simulink model "reachout_demo_PERTURB"  (R2013a)
settings: Solver=ode4  SolverMode=SingleTasking  StartTime=0.0  StopTime=inf  FixedStep=0.0005  RelTol=1e-3
StartFcn:
  |  warndlg('Dexterit-E models cannot run under simulation. Please compile your model and run it from within Dexterit-E.');set_param(bdroot,'SimulationCommand','stop')
model workspace (MAT data in the model file):
  col_x = 1
  col_y = 2
  RADIUS_VIS = 3
  RADIUS_LOG = 4
  COLOR_INIT = 5
  COLOR_REACH = 6
  START_TARGET_COL = 1
  END_TARGET_COL = 7
  LOAD_COL = 8
  DELAY_HAND_FDBK_ON_COL = 11
  MAXREACHTIME_COL = 14
  DELAY_POSTTRIAL_COL = 16
  HAND_FDBK_CNTL_COL = 17
  E_HAND_FDBK_ON = 10
  E_HAND_FDBK_OFF = 11
  WAIT_AT_1stTARGET_COL = 12
  RNDM_WAIT_AT_1stTARGET_COL = 13
  WAIT_AT_2ndTARGET_COL = 15
  X_COL = 1
  Y_COL = 2
  RISE_FALL_COL = 3
  DURATION_COL = 4
  BKIN_STEP_TIME = 0.0005
  TARGET_LABEL = 7
  LABEL_COLOR = 8
  LABEL_SIZE = 9
  GRASP_TARGET = 10
  N_TO_M_GRASP_TAR = 1
  WARNING_COL = 4
  START_FLAG_COL = 6
  TITLE_COL = 5
  E_HOLD_FORCE_1 = 1
  E_HOLD_FORCE_2 = 2
  E_HOLD_1_SUCCESS = 3
  E_HOLD_2_SUCCESS = 4
  E_HOLD_1_FAIL = 5
  E_HOLD_2_FAIL = 6
  E_FORCE_1_LARGER = 7
  E_FORCE_2_LARGER = 8
  E_NOT_HOLDING = 9
  ANSWER_FORCE_1_COL = 2
  ANSWER_FORCE_2_COL = 3
  TIME_TO_ANSWER_COL = 18
  TIME_TO_FAILURE_COL = 19
  CURSOR_OPACITY = 2
  LOAD_1_MAG_COL = 9
  LOAD_2_MAG_COL = 10
  E_LOAD_MAG_1_FIRST = 12
  E_LOAD_MAG_2_FIRST = 13
  GRASP_TARGET_TOLERANCE = 11
undefined symbols (not defined in the file or in its folder): slselsubs
libraries: xpclib x6, Video x6, General x3, KINARM_EP_loads x2, KINARM_general x2, KINARM_IO x1, KINARM_loads x1
CloseFcn:
  | rtwprivate ssgencode ModelCloseRequest b2lab2d
settings Model: ModifiedComment=chris -- Wed Feb 16 09:18:30 2005 -- Version 1.1384  ModifiedHistory=Feb 16/05 - Add error repeat, add offset ramp  ExtModeArmWhenConnect=off  ExtModeLogAll=off  BufferReuse=off  Creator=Chris Grebeldinger  LastModifiedBy=BKIN TECHNOLOGIES
settings DataIOCC: LimitDataPoints=off  SignalLoggingSaveFormat=ModelDataLogs  SaveOutput=off  SaveTime=off  SignalLoggingName=sigsOut
settings OptimizationCC: BlockReduction=off  BooleanDataType=off  OptimizeBlockIOStorage=off  BufferReuse=off  ExpressionFolding=off  ExpressionDepthLimit=2147483647  FoldNonRolledExpr=off  LocalBlockOutputs=off  InitFltsAndDblsToZero=on
settings DebuggingCC: SaveWithParameterizedLinksMsg=none  SignalResolutionControl=TryResolveAllWithWarning  SolverPrmCheckMsg=none  MultiTaskDSMMsg=warning  MultiTaskCondExecSysMsg=none  FcnCallInpInsideContextMsg=UseLocalSettings  StrictBusMsg=None
settings HardwareCC: ProdIntDivRoundTo=Zero  ProdEndianess=LittleEndian  ProdHWDeviceType=Generic->32-bit x86 compatible  TargetHWDeviceType=32-bit Generic
settings RTWCC: SystemTargetFile=xpctarget.tlc  TemplateMakefile=xpc_default_tmf  Description=xPC Target  ProcessScript=xpctarget_make_rtw_hook  IncludeERTFirstTime=on  RTWCompilerOptimization=On
settings CodeAppCC: MaxIdLength=63
settings xpcTargetCC: TargetFcnLib=ansi_tfl_tmw.mat  CodeReplacementLibrary=XPC_BLAS  ParMdlRefBuildCompliant=on  ConcurrentExecutionCompliant=on  CombineSignalStateStructs=off  MATLABClassNameForMDSCustomization=xpcAperiodicCustomization  GRTInterface=on  GenerateAllocFcn=off  xPCTaskExecutionProfile=off  xPCRL32EventNumber=5000  xPCisDownloadable=off  xPCLoadParamSetFile=off  xPCConcurrentTasks=off  xPCEnableSFAnimation=off

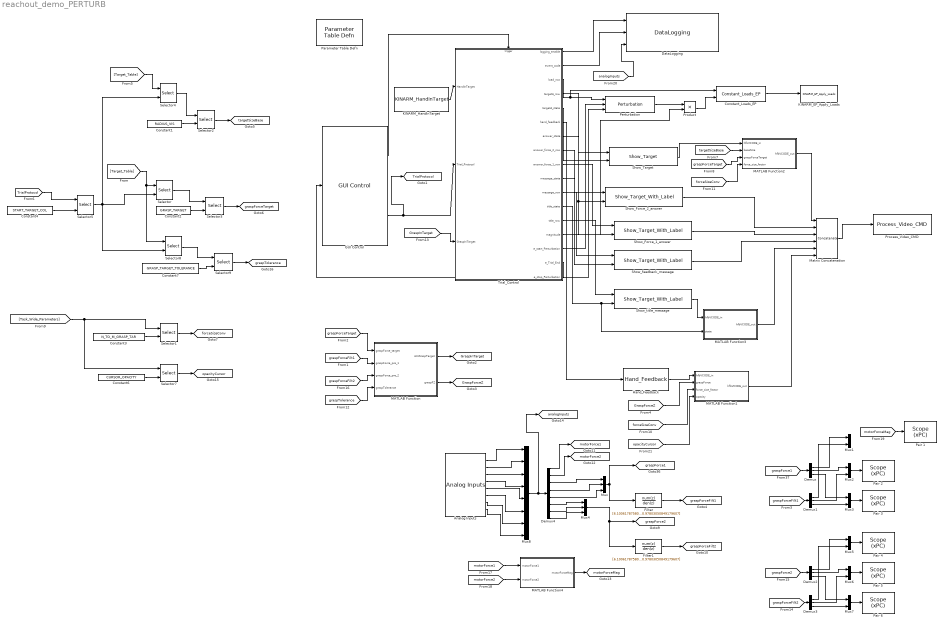
== system reachout_demo_PERTURB ==
  Analog Inputs : KINARM_IO/Analog Inputs  channel=[1,2,5,6,7,8,9,10]  range=[5]  coupling=[0]  scantime6071e=1.28e-5  scantime6229=5e-6  sampletime=0.001  slot=-1  oscantime6071e=0
  Constant1 : Constant  Value=RADIUS_VIS
  Constant2 : Constant  Value=GRASP_TARGET
  Constant3 : Constant  Value=N_TO_M_GRASP_TAR
  Constant4 : Constant  Value=START_TARGET_COL
  Constant6 : Constant  Value=CURSOR_OPACITY
  Constant7 : Constant  Value=GRASP_TARGET_TOLERANCE
  Constant_Loads_EP : KINARM_EP_loads/Constant_Loads_EP  use_dom_hand=on  loadcol=[X_COL Y_COL]  source=port  scaling=1  use_LH_coord=off
  DataLogging : General/DataLogging  log_event_codes=on  log_analog_inputs=on
      link override Poll KINARM/EPTorqueCMD: GotoTag=KINARMEPTorqueCMD
      link override Poll KINARM/TorqueCMD: GotoTag=KINARMTorqueCMD
      link override Poll KINARM/ZeroTorque: Value=[0 0 0 0]
  Demux{,1..3} (4 alike) : Demux  Outputs=3
  Demux4 : Demux  Outputs=8
  Filter : DiscreteFilter  Tag=BlockMethodSubSystem  Numerator=[6.1006178758066243e-05 0.00012201235751613249 6.1006178758066243e-05]  Denominator=[1 -1.9777864837767638 0.97803050849179607]  a0EqualsOne=on
  Filter1 : DiscreteFilter  Tag=BlockMethodSubSystem  Numerator=[6.1006178758066243e-05 0.00012201235751613249 6.1006178758066243e-05]  Denominator=[1 -1.9777864837767638 0.97803050849179607]  a0EqualsOne=on
  GUI Control : General/GUI Control  target_type_str=Circle  Target_Type=1  XYcols=[1 2]  Vcols=3  Lcols=4  indices_padding=[0 0 0 0;0 0 0 0]  task_version=1.0  show_repeat_trial_flag=off
  Hand_Feedback : KINARM_general/Hand_Feedback  feedback_cntl_src=status only
  KINARM_EP_Apply_Loads : KINARM_EP_loads/KINARM_EP_Apply_Loads  up_duration=1500  down_duration=1500  max_force=60
  KINARM_HandInTarget : KINARM_general/KINARM_HandInTarget  use_dominant_hand=on  target_type=Circle  num_states=1  attribcol1=[RADIUS_LOG]  attribcol2=[4]  attribcol3=[5]  attribcol4=[6]  attribcol5=[0]
  MATLAB Function : MATLAB Function  TreatAsAtomicUnit=on
  MATLAB Function1 : MATLAB Function  TreatAsAtomicUnit=on
  MATLAB Function2 : MATLAB Function  TreatAsAtomicUnit=on
  MATLAB Function3 : MATLAB Function  TreatAsAtomicUnit=on
  MATLAB Function4 : MATLAB Function  TreatAsAtomicUnit=on
  Matrix Concatenation : Concatenate  NumInputs=6  Mode=Multidimensional array
  Mux : Mux  Inputs=3
  Mux{1..3,5..7} (6 alike) : Mux  Inputs=2
  Mux4 : Mux  Inputs=3
  Mux8 : Mux  Inputs=8
  Pair 1 : xpclib/Misc./Scope (xPC)   Priority=4  scopeno=1  scopetype=Target  autostart=on  viewmode=Graphical rolling  formatstr='%15.6f'  grid=on  ylimits=[-1,1]  nosamples=1000  noprepostsamples=0  interleave=5  triggermode=FreeRun  triggersignal=1  trigsignalfromport=off  triggerlevel=0.0  triggerslope=Either  triggerscope=1  triggersample=0  filename=data.dat  mode=Lazy  writesize=512  autorestart=off  dynamicfilemode=off  maxwritefilesize=512*1024^2
  Pair 2 : xpclib/Misc./Scope (xPC)   Priority=4  scopeno=2  scopetype=Target  autostart=on  viewmode=Graphical rolling  formatstr='%15.6f'  grid=on  ylimits=[-1,1]  nosamples=1000  noprepostsamples=0  interleave=5  triggermode=FreeRun  triggersignal=1  trigsignalfromport=off  triggerlevel=0.0  triggerslope=Either  triggerscope=1  triggersample=0  filename=data.dat  mode=Lazy  writesize=512  autorestart=off  dynamicfilemode=off  maxwritefilesize=512*1024^2
  Pair 3 : xpclib/Misc./Scope (xPC)   Priority=4  scopeno=3  scopetype=Target  autostart=on  viewmode=Graphical rolling  formatstr='%15.6f'  grid=on  ylimits=[-1,1]  nosamples=1000  noprepostsamples=0  interleave=5  triggermode=FreeRun  triggersignal=1  trigsignalfromport=off  triggerlevel=0.0  triggerslope=Either  triggerscope=1  triggersample=0  filename=data.dat  mode=Lazy  writesize=512  autorestart=off  dynamicfilemode=off  maxwritefilesize=512*1024^2
  Pair 4 : xpclib/Misc./Scope (xPC)   Priority=4  scopeno=4  scopetype=Target  autostart=on  viewmode=Graphical rolling  formatstr='%15.6f'  grid=on  ylimits=[-1,1]  nosamples=1000  noprepostsamples=0  interleave=5  triggermode=FreeRun  triggersignal=1  trigsignalfromport=off  triggerlevel=0.0  triggerslope=Either  triggerscope=1  triggersample=0  filename=data.dat  mode=Lazy  writesize=512  autorestart=off  dynamicfilemode=off  maxwritefilesize=512*1024^2
  Pair 5 : xpclib/Misc./Scope (xPC)   Priority=4  scopeno=5  scopetype=Target  autostart=on  viewmode=Graphical rolling  formatstr='%15.6f'  grid=on  ylimits=[-1,1]  nosamples=1000  noprepostsamples=0  interleave=5  triggermode=FreeRun  triggersignal=1  trigsignalfromport=off  triggerlevel=0.0  triggerslope=Either  triggerscope=1  triggersample=0  filename=data.dat  mode=Lazy  writesize=512  autorestart=off  dynamicfilemode=off  maxwritefilesize=512*1024^2
  Pair 6 : xpclib/Misc./Scope (xPC)   Priority=4  scopeno=6  scopetype=Target  autostart=on  viewmode=Graphical rolling  formatstr='%15.6f'  grid=on  ylimits=[-1,1]  nosamples=1000  noprepostsamples=0  interleave=5  triggermode=FreeRun  triggersignal=1  trigsignalfromport=off  triggerlevel=0.0  triggerslope=Either  triggerscope=1  triggersample=0  filename=data.dat  mode=Lazy  writesize=512  autorestart=off  dynamicfilemode=off  maxwritefilesize=512*1024^2
  Parameter Table Defn : General/Parameter Table Defn  ShowInLibBrowser=0
  Perturbation : KINARM_loads/Perturbation  loadcol=[RISE_FALL_COL DURATION_COL RISE_FALL_COL]
  Process_Video_CMD : Video/Process_Video_CMD
  Product : Product
  Selector : Selector  NumberOfDimensions=2  InputPortWidth=3  IndexOptions=Index vector (port),Select all  Indices=1,-1  OutputSizes=slselsubs([(-2),(-2)],1),slselsubs([(-2),(-2)],2)
  Selector{1..3,7,9} (5 alike) : Selector  NumberOfDimensions=2  InputPortWidth=3  IndexOptions=Select all,Starting index (port)  Indices=[1 3],1  OutputSizes=1,1
  Selector4 : Selector  NumberOfDimensions=2  InputPortWidth=3  IndexOptions=Index vector (port),Select all  Indices=1,-1  OutputSizes=slselsubs([(-2),(-2)],1),slselsubs([(-2),(-2)],2)
  Selector5 : Selector  NumberOfDimensions=2  InputPortWidth=3  IndexOptions=Select all,Index vector (port)  Indices=1,-1  OutputSizes=slselsubs([(-2),(-2)],1),slselsubs([(-2),(-2)],2)
  Selector8 : Selector  NumberOfDimensions=2  InputPortWidth=3  IndexOptions=Index vector (port),Select all  Indices=1,-1  OutputSizes=slselsubs([(-2),(-2)],1),slselsubs([(-2),(-2)],2)
  Show_Force_1_answer : Video/Show_Target_With_Label  target_type=Circle  num_states=1  attribcol1=[5 5 0 3 7 8 9]  attribcol2=[6 6 0 3 0 0 0]  attribcol3=[0 0 0 0 0 0 0]  attribcol4=[0 0 0 0 0 0 0]  attribcol5=[0 0 24 0 0 0 0]  stateindices_padding=[0 0 0 0;0 0 0 0;0 0 0 0;0 0 0 0;0 0 0 0]  source=dialog  opacity=100  target_display=Both subject and operator displays
  Show_Force_2_answer : Video/Show_Target_With_Label  target_type=Circle  num_states=1  attribcol1=[5 5 0 3 7 8 9]  attribcol2=[6 6 0 3 0 0 0]  attribcol3=[0 0 0 0 0 0 0]  attribcol4=[0 0 0 0 0 0 0]  attribcol5=[0 0 24 0 0 0 0]  stateindices_padding=[0 0 0 0;0 0 0 0;0 0 0 0;0 0 0 0;0 0 0 0]  source=dialog  opacity=100  target_display=Both subject and operator displays
  Show_Target : Video/Show_Target  target_type=Circle  num_states=2  attribcol1=[0 COLOR_INIT -1 RADIUS_VIS]  attribcol2=[0 COLOR_REACH -1 RADIUS_VIS]  attribcol3=[0 0 0 0]  attribcol4=[0 0 0 0]  attribcol5=[0 0 24 0]  stateindices_padding=[0 0 0 0 0 0 0;0 0 0 0 0 0 0;0 0 0 0 0 0 0;0 0 0 0 0 0 0;0 0 0 0 0 0 0]  source=dialog  opacity=100  target_display=Both subject and operator displays  num_col=4
  Show_feedback_message : Video/Show_Target_With_Label  target_type=Circle  num_states=1  attribcol1=[5 5 0 3 7 8 9]  attribcol2=[6 6 0 3 0 0 0]  attribcol3=[0 0 0 0 0 0 0]  attribcol4=[0 0 0 0 0 0 0]  attribcol5=[0 0 24 0 0 0 0]  stateindices_padding=[0 0 0 0;0 0 0 0;0 0 0 0;0 0 0 0;0 0 0 0]  source=dialog  opacity=100  target_display=Both subject and operator displays
  Show_title_message : Video/Show_Target_With_Label  target_type=Circle  num_states=4  attribcol1=[5 5 0 3 7 8 9]  attribcol2=[5 5 0 3 7 8 9]  attribcol3=[5 5 0 3 7 8 9]  attribcol4=[5 5 0 3 7 8 9]  attribcol5=[0 0 24 0 0 0 0]  stateindices_padding=[0 0 0 0;0 0 0 0;0 0 0 0;0 0 0 0;0 0 0 0]  source=dialog  opacity=100  target_display=Both subject and operator displays
  Trial_Control : Stateflow chart  TreatAsAtomicUnit=on
  tag scope: GraspForceZ=global, GraspInTarget=global, TrialProtocol=global, analogInputs=global, forceSizeConv=global, graspForce1=global, graspForce2=global, graspForceFilt1=global, graspForceFilt2=global, graspForceTarget=global, graspTolerance=global, motorForce1=global, motorForce2=global, motorForceMag=global, opacityCursor=global, targetSizeBase=global
  wires:
  KINARM_HandInTarget/1 -> Trial_Control/1(HandInTarget)
  Trial_Control/16(e_Trial_End) -> GUI Control/1
  GUI Control/1 -> Trial_Control/Trigger
  Trial_Control/5(targetA_state) -> Show_Target/2
  Matrix Concatenation/1 -> Process_Video_CMD/1
  Trial_Control/6(hand_feedback) -> Hand_Feedback/1
  Constant_Loads_EP/1 -> KINARM_EP_Apply_Loads/1
  Trial_Control/3(load_row) -> Perturbation/1, Constant_Loads_EP/1
  Perturbation/1 -> Product/1
  Trial_Control/15(e_start_Perturbation) -> Perturbation/2
  Trial_Control/1(logging_enable) -> DataLogging/1
  Trial_Control/2(event_code) -> DataLogging/2
  Show_Force_1_answer/1 -> Matrix Concatenation/3
  Trial_Control/7(answer_state) -> Show_Force_1_answer/2, Show_Force_2_answer/2
  Show_Force_2_answer/1 -> Matrix Concatenation/2
  Trial_Control/8(answer_force_2_row) -> Show_Force_2_answer/1
  Trial_Control/9(answer_force_1_row) -> Show_Force_1_answer/1
  Analog Inputs/3 -> Mux8/3
  Analog Inputs/4 -> Mux8/4
  Analog Inputs/5 -> Mux8/5
  Mux/1 -> [graspForce1], Filter/1
  [graspForce1] -> Demux/1
  Demux/1 -> Mux1/1
  Demux/2 -> Mux2/1
  Demux/3 -> Mux3/1
  [graspForceFilt1] -> MATLAB Function/2(graspForce_pre_1)
  GUI Control/2 -> [TrialProtocol], Trial_Control/2(Trial_Protocol)
  MATLAB Function/1(isInGraspTarget) -> [GraspInTarget]
  Hand_Feedback/1 -> MATLAB Function1/1(hfbVCODE_in)
  MATLAB Function/2(graspFZ) -> [GraspForceZ]
  [GraspForceZ] -> MATLAB Function1/2(graspForce)
  MATLAB Function1/1(hfbVCODE_out) -> Matrix Concatenation/6
  Filter/1 -> [graspForceFilt1]
  [graspForceFilt1] -> Demux1/1
  Demux1/1 -> Mux1/2
  Demux1/2 -> Mux2/2
  Demux1/3 -> Mux3/2
  Mux2/1 -> Pair 2/1
  Mux3/1 -> Pair 3/1
  Show_Target/1 -> MATLAB Function2/1(hfbVCODE_in)
  MATLAB Function2/1(hfbVCODE_out) -> Matrix Concatenation/1
  Constant1/1 -> Selector2/2
  Constant2/1 -> Selector3/2
  Selector2/1 -> [targetSizeBase]
  Selector3/1 -> [graspForceTarget]
  [targetSizeBase] -> MATLAB Function2/2(baseSize)
  [graspForceTarget] -> MATLAB Function2/3(graspForceTarget)
  [graspForceTarget] -> MATLAB Function/1(graspForce_target)
  Constant3/1 -> Selector1/2
  Selector1/1 -> [forceSizeConv]
  [forceSizeConv] -> MATLAB Function1/3(force_size_factor)
  [forceSizeConv] -> MATLAB Function2/4(force_size_factor)
  Selector/1 -> Selector3/1
  Selector4/1 -> Selector2/1
  [Target_Table] -> Selector4/1
  [GraspInTarget] -> Trial_Control/3(GraspInTarget)
  Trial_Control/4(targetA_row) -> Show_Target/1
  Constant4/1 -> Selector5/2
  [TrialProtocol] -> Selector5/1
  Trial_Control/10(message_state) -> Show_feedback_message/2
  Show_feedback_message/1 -> Matrix Concatenation/4
  Trial_Control/11(message_row) -> Show_feedback_message/1
  [graspTolerance] -> MATLAB Function/4(graspTolerance)
  Mux4/1 -> Filter1/1, [graspForce2]
  Filter1/1 -> [graspForceFilt2]
  Analog Inputs/6 -> Mux8/6
  Analog Inputs/7 -> Mux8/7
  Analog Inputs/8 -> Mux8/8
  [graspForce2] -> Demux2/1
  Demux2/1 -> Mux5/1
  Demux2/2 -> Mux6/1
  Demux2/3 -> Mux7/1
  [graspForceFilt2] -> Demux3/1
  Mux5/1 -> Pair 4/1
  Demux3/1 -> Mux5/2
  Demux3/2 -> Mux6/2
  Demux3/3 -> Mux7/2
  Mux6/1 -> Pair 5/1
  Mux7/1 -> Pair 6/1
  [graspForceFilt2] -> MATLAB Function/3(graspForce_pre_2)
  Trial_Control/12(title_state) -> MATLAB Function3/2(state), Show_title_message/2
  Trial_Control/13(title_row) -> Show_title_message/1
  Show_title_message/1 -> MATLAB Function3/1(hfbVCODE_in)
  MATLAB Function3/1(hfbVCODE_out) -> Matrix Concatenation/5
  Analog Inputs/1 -> Mux8/1
  Analog Inputs/2 -> Mux8/2
  [motorForce1] -> MATLAB Function4/1(motorForce1)
  [motorForce2] -> MATLAB Function4/2(motorForce2)
  MATLAB Function4/1(motorForceMag) -> [motorForceMag]
  [motorForceMag] -> Pair 1/1
  Trial_Control/17(e_stop_Perturbation) -> Perturbation/3
  Mux8/1 -> [analogInputs], Demux4/1
  Demux4/1 -> [motorForce1]
  Demux4/2 -> [motorForce2]
  Demux4/3 -> Mux/1
  Demux4/4 -> Mux/2
  Demux4/5 -> Mux/3
  Demux4/6 -> Mux4/1
  Demux4/7 -> Mux4/2
  Demux4/8 -> Mux4/3
  [analogInputs] -> DataLogging/3
  Constant6/1 -> Selector7/2
  Selector7/1 -> [opacityCursor]
  [Task_Wide_Parameters] -> Selector7/1, Selector1/1
  [opacityCursor] -> MATLAB Function1/4(opacity)
  Product/1 -> Constant_Loads_EP/2
  Trial_Control/14(magnitude) -> Product/2
  Constant7/1 -> Selector9/2
  Selector9/1 -> [graspTolerance]
  [Target_Table] -> Selector8/1, Selector/1
  Selector8/1 -> Selector9/1
  Selector5/1 -> Selector8/2, Selector/2, Selector4/2

== stateflow chart reachout_demo_PERTURB/Trial_Control ==
  settings: sampleTime=0.001
  state Initialize/
    // Turn off both targets, set hand_feedback on
    targetA_state=0;
    answer_state = 0;
    message_state = 0;
    title_state =0;
    hand_feedback=1;
    title_row = Trial_Protocol[TITLE_COL];
  state Main_Trial
    state SetLoadOrder1/
      magnitude_1 = Trial_Protocol[LOAD_1_MAG_COL];
      magnitude_2 = Trial_Protocol[LOAD_2_MAG_COL];
      event_code = E_LOAD_MAG_1_FIRST;
    state ShuffleLoads/
      rand_num = rand()/RAND_MAX;
      logging_enable = 1;
    state SetLoadOrder2/
      magnitude_1 = Trial_Protocol[LOAD_2_MAG_COL];
      magnitude_2 = Trial_Protocol[LOAD_1_MAG_COL];
      event_code = E_LOAD_MAG_2_FIRST;
    state FirstTargetOn/
      // Turn on first target, set loading conditions, enable data logging, wait for specified delay or until hand-is-in-target
      logging_enable = 0;
      targetA_row = Trial_Protocol[START_TARGET_COL];
      targetA_state=1;
      magnitude = magnitude_1;
      load_row = Trial_Protocol[LOAD_COL];
      tickCount =Trial_Protocol[DELAY_HAND_FDBK_ON_COL];
    state HandFeedbackOn/
      // Turn on handfeedback
      hand_feedback=1;
      targetA_state = 1;
    state StayAtFirstTarget/
      // change the first target state, log an event, wait for specified (randomized) period of time.  Hand must STAY in target for specified time.
      logging_enable = 1;
      message_state = 0;
      title_state = 0;
      event_code = E_HOLD_FORCE_1;
      targetA_state = 2;
      tickCount = Trial_Protocol[WAIT_AT_1stTARGET_COL]+Trial_Protocol[RNDM_WAIT_AT_1stTARGET_COL]*rand()/RAND_MAX;
    state FailedHold1/
      // Show warning to go to target
      message_state = 0;
      title_state = 4;
      targetA_state = 1;
      e_stop_Perturbation;
      event_code = E_HOLD_1_FAIL;
    state DeliverForce1/
      // Delay one step for E_HAND_FEEDBACK_OFF to
      // be processed prior to next state
      tickCount =Trial_Protocol[MAXREACHTIME_COL];
      title_state = 1;
      e_start_Perturbation;
    state ForceHold1//
      state OutOfTarget/
        // Show warning to go to target
        tickCount_fail = Trial_Protocol[TIME_TO_FAILURE_COL];
        message_state = 1;
        message_row = Trial_Protocol[WARNING_COL];
        targetA_state = 1;
      state Deliver1stLoad/
        // Deliver load, if hand leaves target (position or grasp force), go to warning state
        //event_code = E_FIRST_LOAD_ON;
        targetA_state = 2;
        message_state = 1;
        message_row = Trial_Protocol[START_FLAG_COL];
        hand_feedback = 0;
      Main_Trial.ForceHold1.Deliver1stLoad -> Main_Trial.ForceHold1.OutOfTarget : [HandInTarget[targetA_row]==0 || GraspInTarget == 0]/
          | event_code = E_NOT_HOLDING;
      Main_Trial.ForceHold1.OutOfTarget -> Main_Trial.ForceHold1.Deliver1stLoad [order 2] : [HandInTarget[targetA_row]==1 && GraspInTarget == 1]
    state NotInTarget/
      targetA_state = 1;
    state StayAtSecondTarget/
      // Deliver 2nd load
      message_state = 0;
      title_state = 0;
      targetA_state = 2;
      magnitude = magnitude_2;
      load_row = Trial_Protocol[LOAD_COL];
      event_code = E_HOLD_FORCE_2
      tickCount =Trial_Protocol[WAIT_AT_1stTARGET_COL]+Trial_Protocol[RNDM_WAIT_AT_1stTARGET_COL]*rand()/RAND_MAX;
    state FailedHold2/
      // Show warning to go to target
      message_state = 0;
      title_state = 4;
      targetA_state = 1;
      e_stop_Perturbation;
      event_code = E_HOLD_2_FAIL;
    state DeliverForce2/
      // Deliver 2nd load
      //event_code = E_SECOND_LOAD_ON;
      tickCount =Trial_Protocol[MAXREACHTIME_COL];
      title_state = 2;
      e_start_Perturbation;
    state ForceHold2//
      state OutOfTarget/
        // Show warning to go to target
        tickCount_fail = Trial_Protocol[TIME_TO_FAILURE_COL];
        message_state = 1;
        message_row = Trial_Protocol[WARNING_COL];
        targetA_state = 1;
      state Deliver1stLoad/
        // Deliver load, if hand leaves target (position or grasp force), go to warning state
        //event_code = E_FIRST_LOAD_ON;
        targetA_state = 2;
        message_state = 1;
        message_row = Trial_Protocol[START_FLAG_COL];
        hand_feedback = 0;
      Main_Trial.ForceHold2.Deliver1stLoad -> Main_Trial.ForceHold2.OutOfTarget : [HandInTarget[targetA_row]==0 || GraspInTarget == 0]/
          | event_code = E_NOT_HOLDING;
      Main_Trial.ForceHold2.OutOfTarget -> Main_Trial.ForceHold2.Deliver1stLoad [order 2] : [HandInTarget[targetA_row]==1 && GraspInTarget == 1]
    state ShowAnswerOptions/
      targetA_state = 0;
      message_state = 0;
      answer_state = 1;
      hand_feedback = 1;
      title_state = 3;
      answer_force_1_row = Trial_Protocol[ANSWER_FORCE_1_COL];
      answer_force_2_row = Trial_Protocol[ANSWER_FORCE_2_COL];
    state HoldAnswerForce1Larger/
      tickCount = Trial_Protocol[TIME_TO_ANSWER_COL];
    state HoldAnswerForce2Larger/
      tickCount = Trial_Protocol[TIME_TO_ANSWER_COL];
    state EndOfTrial/
      // Wait for a specified period of time,
      tickCount =Trial_Protocol[DELAY_POSTTRIAL_COL];
    (junction 174) -> SetLoadOrder1 [order 1] : [rand_num >= 0.5]
    SetLoadOrder1 -> FirstTargetOn
    ShuffleLoads -> (junction 174)
    (junction 174) -> SetLoadOrder2 [order 2] : [rand_num < 0.5]
    SetLoadOrder2 -> FirstTargetOn
    FirstTargetOn -> HandFeedbackOn [order 2] : [HandInTarget[targetA_row]==1]
    FirstTargetOn -> HandFeedbackOn [order 1] : after(tickCount, e_clk)
    StayAtFirstTarget -> HandFeedbackOn [order 2] : [HandInTarget[targetA_row]==0 || GraspInTarget == 0]
    HandFeedbackOn -> StayAtFirstTarget : [HandInTarget[targetA_row]==1 && GraspInTarget == 1]
    FailedHold1 -> StayAtFirstTarget : [HandInTarget[targetA_row]==1 && GraspInTarget == 1]
    StayAtFirstTarget -> (junction 27) [order 1] : after(tickCount, e_clk)
        | {hand_feedback=Trial_Protocol[HAND_FDBK_CNTL_COL]}
        | // Turn handfeedback on or off (from Trial Protocol Table)
    (junction 27) -> DeliverForce1 [order 1] : [hand_feedback==0]/
        | // if hand feedback is turned off, log an event
        | event_code=E_HAND_FDBK_OFF;
    (junction 27) -> DeliverForce1 [order 2]
    ForceHold1 -> NotInTarget : [after(tickCount, e_clk)]/
        | event_code = E_HOLD_1_SUCCESS
    StayAtSecondTarget -> NotInTarget [order 2] : [HandInTarget[targetA_row]==0 || GraspInTarget == 0]
    NotInTarget -> StayAtSecondTarget : [HandInTarget[targetA_row]==1 && GraspInTarget == 1]
    FailedHold2 -> StayAtSecondTarget : [HandInTarget[targetA_row]==1 && GraspInTarget == 1]
    StayAtSecondTarget -> DeliverForce2 [order 1] : after(tickCount, e_clk)
    ForceHold2 -> ShowAnswerOptions : [after(tickCount, e_clk)]/
        | event_code = E_HOLD_2_SUCCESS
    HoldAnswerForce2Larger -> ShowAnswerOptions [order 1] : [HandInTarget[answer_force_2_row]==0]
    HoldAnswerForce1Larger -> ShowAnswerOptions [order 2] : [HandInTarget[answer_force_1_row]==0]
    ShowAnswerOptions -> HoldAnswerForce1Larger [order 2] : [HandInTarget[answer_force_1_row]==1]
    ShowAnswerOptions -> HoldAnswerForce2Larger [order 1] : [HandInTarget[answer_force_2_row]==1]
    HoldAnswerForce1Larger -> EndOfTrial [order 1] : [after(tickCount,e_clk)]/
        | event_code = E_FORCE_1_LARGER
    HoldAnswerForce2Larger -> EndOfTrial [order 2] : [after(tickCount,e_clk)]/
        | event_code = E_FORCE_2_LARGER
    Main_Trial.ForceHold1.OutOfTarget -> FailedHold1 [order 1] : after(tickCount_fail,e_clk)
    Main_Trial.ForceHold2.OutOfTarget -> FailedHold2 [order 1] : after(tickCount_fail,e_clk)
    DeliverForce1 -> Main_Trial.ForceHold1.Deliver1stLoad
    DeliverForce2 -> Main_Trial.ForceHold2.Deliver1stLoad
  state Inter_Trial_State/
    // send e_Trial_End event
    e_Trial_End;
    // turn off both targets
    // stop data logging
    targetA_state=0;
    answer_state = 0;
    logging_enable = 0;
    title_state = 0;
  (default) -> Initialize
  Initialize -> ShuffleLoads
  Inter_Trial_State -> ShuffleLoads : after(tickCount, e_clk)
  Main_Trial -> Inter_Trial_State : e_ExitTrialNow/
      | // if e_ExitTrialNow event occurs,
      | tickCount=1;
  EndOfTrial -> Inter_Trial_State
  data: HandInTarget input double; logging_enable output boolean; event_code output uint16 [0..] =0; load_row output [1..32]; Trial_Protocol input double; targetA_row output [1..32]; targetA_state output double; tickCount local double; hand_feedback output double; RAND_MAX constant double =32767; answer_state output double; answer_force_2_row output [1..32]; answer_force_1_row output; GraspInTarget input boolean; message_state output double; message_row output double; tickCount_fail local double; title_state output double; title_row output double; magnitude output double; magnitude_1 local double; magnitude_2 local double; rand_num local double
  data load_row settings: description=current index into the loadtable
  data targetA_row settings: description=index of the row currently being used in the TargetTable
  data answer_force_2_row settings: description=current index into the loadtable
  events: e_start_Perturbation output EITHER_EDGE_EVENT; e_clk input RISING_EDGE_EVENT; e_ExitTrialNow input EITHER_EDGE_EVENT; e_Trial_End output EITHER_EDGE_EVENT; e_stop_Perturbation output EITHER_EDGE_EVENT

== matlab function reachout_demo_PERTURB/MATLAB Function ==
  data: graspForce_target input; graspForce_pre_1 input; graspForce_pre_2 input; isInGraspTarget output; graspFZ output; graspTolerance input
function [isInGraspTarget,graspFZ] = isInGraspForceTarget(graspForce_target,graspForce_pre_1,graspForce_pre_2,graspTolerance)
% isInGraspTarget - 1: Is within grasp target tolerance
% isInGraspTarget - 2: Is below grasp target tolerance
% isInGraspTarget - 3: Is above grasp target tolerance

graspForce_1 = graspForce_pre_1.*[250;250;500]/5;
graspForce_2 = graspForce_pre_2.*[250;250;500]/5;

graspFZ = min([graspForce_1(3) graspForce_2(3)]);

low_tol = (100 - graspTolerance)/100;
high_tol = (100 + graspTolerance)/100;

isInGraspTarget = (graspFZ >= low_tol*graspForce_target)&(graspFZ <= high_tol*graspForce_target);

end

== matlab function reachout_demo_PERTURB/MATLAB Function1 ==
  data: hfbVCODE_in input; graspForce input; hfbVCODE_out output; force_size_factor input; opacity input
function hfbVCODE_out = HandFeedbackSizeandOpacity(hfbVCODE_in,graspForce,force_size_factor,opacity)

% force_size_factor = 0.005; % m/N

hfbVCODE_in(:,9) = opacity;
hfbVCODE_in(:,10) = 0.005+abs(graspForce)*force_size_factor; % [m/N]
hfbVCODE_out = hfbVCODE_in;

end

== matlab function reachout_demo_PERTURB/MATLAB Function2 ==
  data: hfbVCODE_in input; baseSize input; hfbVCODE_out output; graspForceTarget input; force_size_factor input
function hfbVCODE_out = GraspForceTargetSize(hfbVCODE_in,baseSize,graspForceTarget,force_size_factor)
%baseSize is in cm
% force_size_factor = 0.005; % m/N
targetSize = baseSize/100 + graspForceTarget*force_size_factor;

hfbVCODE_in(:,10) = targetSize;
hfbVCODE_out = hfbVCODE_in;

% Remove fill


end

== matlab function reachout_demo_PERTURB/MATLAB Function3 ==
  data: hfbVCODE_in input; state input; hfbVCODE_out output
function hfbVCODE_out = TitleLegend(hfbVCODE_in,state)

VCODE = hfbVCODE_in;

switch state 
    case 1
        VCODE(15) = 49; % 1
        VCODE(16) = 115; % s
        VCODE(17) = 116; % t
        VCODE(18) = 32; % space
        VCODE(19) = 70; % F
        VCODE(20) = 111; % o
        VCODE(21) = 114; % r
        VCODE(22) = 99; % c
        VCODE(23) = 101; % e
    case 2
        VCODE(15) = 50; % 2
        VCODE(16) = 110; % n
        VCODE(17) = 100; % d
        VCODE(18) = 32; % space
        VCODE(19) = 70; % F
        VCODE(20) = 111; % o
        VCODE(21) = 114; % r
        VCODE(22) = 99; % c
        VCODE(23) = 101; % e
    case 3
        VCODE(15) = 87; % W
        VCODE(16) = 104; % h
        VCODE(17) = 97; % a
        VCODE(18) = 116; % t
        VCODE(19) = 32; % space
        VCODE(20) = 102; % f
        VCODE(21) = 111; % o
        VCODE(22) = 114; % r
        VCODE(23) = 99; % c
        VCODE(24) = 101; % e
        VCODE(25) = 32; % space
        VCODE(26) = 119; % w
        VCODE(27) = 97; % a
        VCODE(28) = 115; % s
        VCODE(29) = 32; % space
        VCODE(30) = 108; % l
        VCODE(31) = 97; % a
        VCODE(32) = 114; % r
        VCODE(33) = 103; % g
        VCODE(34) = 101; % e
        VCODE(35) = 114; % r
        VCODE(36) = 63; % ?   
    case 4
         VCODE(15) = 70; % F
        VCODE(16) = 97; % a
        VCODE(17) = 105; % i
        VCODE(18) = 108; % l
        VCODE(19) = 117; % u
        VCODE(20) = 114; % r
        VCODE(21) = 101; % e
end

hfbVCODE_out = VCODE;

end

== matlab function reachout_demo_PERTURB/MATLAB Function4 ==
  data: motorForce1 input; motorForce2 input; motorForceMag output
function motorForceMag = MotorForceMagnitude(motorForce1,motorForce2)

motorForceMag = sqrt(motorForce1.^2 + motorForce2.^2);

end
